simulink model "dcmotor_pid"  (R2024b)
settings: Solver=ode45  StartTime=0.0  StopTime=2  MaxStep=1e-3  RelTol=1e-6
InitFcn:
  | motor_params; apply_scenario;
undefined symbols (not defined in the file): ctrl, motor, scn
libraries: slpidlib x1
Description:
  | v0.1 DC motor speed control: PI with 24 V limit and clamping anti-windup.
settings Model: Creator=HP PC  LastModifiedBy=HP PC

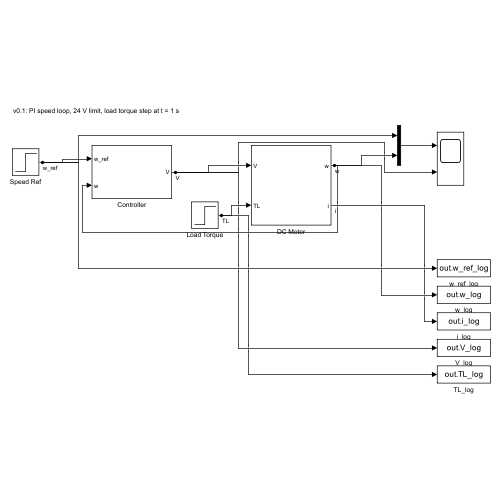
[thumbnail: Simulink's stored preview of the top-level diagram]
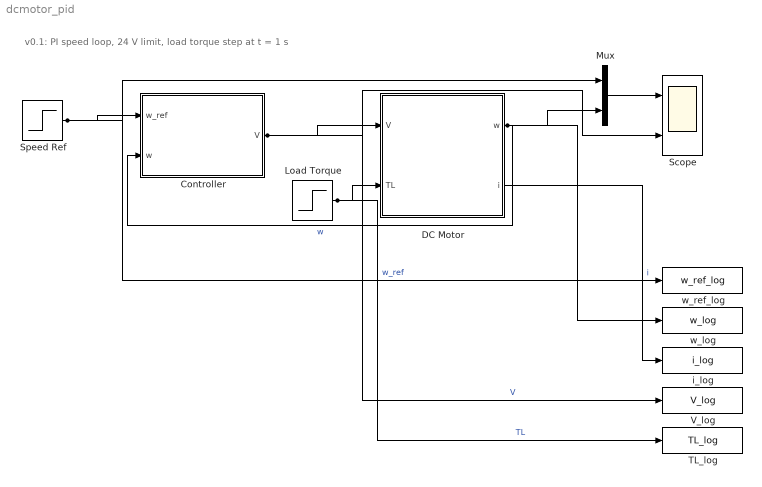
== system dcmotor_pid ==
  note: v0.1: PI speed loop, 24 V limit, load torque step at t = 1 s
  Controller : Subsystem
  DC Motor : Subsystem
  Load Torque : Step  Time=scn.t_load  After=scn.TL  SampleTime=0
  Mux : Mux  Inputs=2
  Scope : Scope  NumInputPorts=2
  Speed Ref : Step  Time=scn.t_ref  After=scn.w_ref  SampleTime=0
  TL_log : ToWorkspace  VariableName=TL_log  SaveFormat=Timeseries  SampleTime=-1
  V_log : ToWorkspace  VariableName=V_log  SaveFormat=Timeseries  SampleTime=-1
  i_log : ToWorkspace  VariableName=i_log  SaveFormat=Timeseries  SampleTime=-1
  w_log : ToWorkspace  VariableName=w_log  SaveFormat=Timeseries  SampleTime=-1
  w_ref_log : ToWorkspace  VariableName=w_ref_log  SaveFormat=Timeseries  SampleTime=-1
  wires:
  Speed Ref/1 -> Controller/1(w_ref), Mux/1, w_ref_log/1  "w_ref"
  Controller/1(V) -> DC Motor/1(V), Scope/2, V_log/1  "V"
  Load Torque/1 -> DC Motor/2(TL), TL_log/1  "TL"
  DC Motor/1(w) -> Controller/2(w), Mux/2, w_log/1  "w"
  Mux/1 -> Scope/1
  DC Motor/2(i) -> i_log/1  "i"

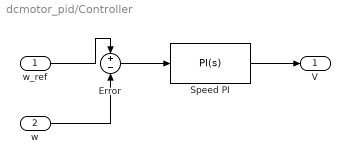
== system dcmotor_pid/Controller ==
  w_ref : Inport
  w : Inport  Port=2
  Error : Sum  Inputs=+-
  Speed PI : slpidlib/PID Controller  Controller=PI  Form=Parallel  TimeDomain=Continuous-time  UseExternalTs=off  SampleTime=-1  IntegratorMethod=Forward Euler  FilterMethod=Forward Euler  ControllerParametersSource=internal  P=ctrl.Kp  I=ctrl.Ki  UseKiTs=off  D=0  UseExternalDerivativeSource=off  N=100  UseFilter=on  TunerSelectOption=Transfer Function Based (PID Tuner App)  InitialConditionSource=internal  InitialConditionForIntegrator=0  InitialConditionForFilter=0  DifferentiatorICPrevScaledInput=0  ExternalReset=none  TrackingMode=off  Kt=1  LimitOutput=on  SatLimitsSource=internal  UpperSaturationLimit=ctrl.Vmax  LowerSaturationLimit=-ctrl.Vmax  LinearizeAsGain=on  AntiWindupMode=clamping  Kb=1  LimitIntegrator=off  UpperIntegratorSaturationLimit=inf  LowerIntegratorSaturationLimit=-inf  POutMin=[]  POutMax=[]  IOutMin=[]  IOutMax=[]  DOutMin=[]  DOutMax=[]  NOutMin=[]  NOutMax=[]  SumOutMin=[]  SumOutMax=[]  SaturationOutMin=[]  SaturationOutMax=[]  PParamMin=[]  PParamMax=[]  IParamMin=[]  IParamMax=[]  DParamMin=[]  DParamMax=[]  NParamMin=[]  NParamMax=[]  KbParamMin=[]  KbParamMax=[]  KtParamMin=[]  KtParamMax=[]  KbOutMin=[]  KbOutMax=[]  KtOutMin=[]  KtOutMax=[]  IntegratorOutMin=[]  IntegratorOutMax=[]  FilterOutMin=[]  FilterOutMax=[]  SumI1OutMin=[]  SumI1OutMax=[]  SumI2OutMin=[]  SumI2OutMax=[]  SumI3OutMin=[]  SumI3OutMax=[]  SumI4OutMin=[]  SumI4OutMax=[]  SumDOutMin=[]  SumDOutMax=[]  DifferentiatorOutMin=[]  DifferentiatorOutMax=[]  FilterDiffOutCoefMin=[]  FilterDiffOutCoefMax=[]  ReciprocalOutMin=[]  ReciprocalOutMax=[]  SumDenOutMin=[]  SumDenOutMax=[]  SumNumOutMin=[]  SumNumOutMax=[]  DivideOutMin=[]  DivideOutMax=[]  UdiffTsProdOutMin=[]  UdiffTsProdOutMax=[]  NTsProdOutMin=[]  NTsProdOutMax=[]  UintegralTsProdOutMin=[]  UintegralTsProdOutMax=[]  UngainTsProdOutMin=[]  UngainTsProdOutMax=[]  ClampingZeroOutDataTypeStr=Inherit: Inherit via back propagation  ClampingZeroOutMin=[]  ClampingZeroOutMax=[]  FilterDenConstantOutDataTypeStr=Inherit: Inherit via back propagation  FilterDenConstantOutMin=[]  FilterDenConstantOutMax=[]  PCopyOutDataTypeStr=Inherit: Inherit via back propagation  PCopyOutMin=[]  PCopyOutMax=[]  NCopyOutDataTypeStr=Inherit: Inherit via back propagation  NCopyOutMin=[]  NCopyOutMax=[]  IntegratorContinuousStateAttributes=''  IntegratorStateMustResolveToSignalObject=off  IntegratorRTWStateStorageClass=Auto  FilterContinuousStateAttributes=''  FilterStateMustResolveToSignalObject=off  FilterRTWStateStorageClass=Auto  ParallelPVariant=InternalParameters  IdealPVariant=Disabled  IVariant=InternalParameters  DVariant=Disabled  IntegratorVariant=Continuous  SatVariant=Enabled  AWVariant=ContClampingParallel  PCopyVariant=Disabled  TRVariant=Disabled  FdbkBlocksVariant=Forward  IdealPFdbkVariant=Disabled  SatFdbkVariant=Disabled  DerivativeFilterVariant=Disabled  NVariant=Disabled  NCopyVariant=Disabled_SignalSpec  FilterICVariant=Disabled  IntegratorICVariant=InternalICs  ExternalResetVariant=Disabled  TRSumVariant=Passthrough  SumFdbkVariant=Disabled  SumVariant=Sum_PI  TsampFilterVariant=InternalTs  TsampNgainVariant=Passthrough  TsampIntegralVariant=Disabled_SignalSpec  ExternalSaturationOutDataTypeStr=Inherit: Same as second input  DerivativeSourceVariant=Disabled  PreIntVariant=InternalPreInt
  V : Outport
  wires:
  w_ref/1 -> Error/1
  w/1 -> Error/2
  Error/1 -> Speed PI/1
  Speed PI/1 -> V/1

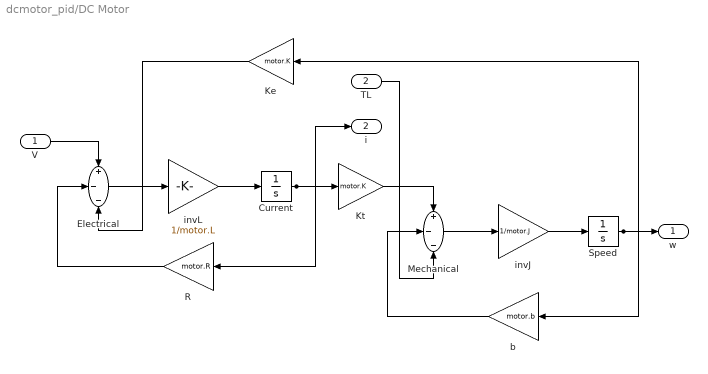
== system dcmotor_pid/DC Motor ==
  V : Inport
  TL : Inport  Port=2
  Current : Integrator  InitialCondition=motor.i0
  Electrical : Sum  Inputs=+--
  Ke : Gain  Gain=motor.K
  Kt : Gain  Gain=motor.K
  Mechanical : Sum  Inputs=+--
  R : Gain  Gain=motor.R
  Speed : Integrator  InitialCondition=motor.w0
  b : Gain  Gain=motor.b
  invJ : Gain  Gain=1/motor.J
  invL : Gain  Gain=1/motor.L
  w : Outport
  i : Outport  Port=2
  wires:
  Ke/1 -> Electrical/3
  V/1 -> Electrical/1
  Kt/1 -> Mechanical/1
  Electrical/1 -> invL/1
  R/1 -> Electrical/2
  invL/1 -> Current/1
  TL/1 -> Mechanical/3
  Current/1 -> R/1, Kt/1, i/1
  Mechanical/1 -> invJ/1
  b/1 -> Mechanical/2
  invJ/1 -> Speed/1
  Speed/1 -> b/1, Ke/1, w/1
